simulink model "Cb_Integral_Control_Observer"  (R2025b)
settings: Solver=ode15s  StartTime=0.0  StopTime=2  RelTol=1e-9  AbsTol=1e-8
undefined symbols (not defined in the file): A11, A12, A21, A22, Bd1, Bd2, Bu1, Bu2, CA_re, CAin_re, CB_re, KH1, KH2, KH3, KH4, Ki1, Ki2, Kin1, Kin2, Kin3, Kin4, L, QH_re, Qin_V_re, T_re, Tc_re, Tin_re
settings Model: Creator=Lenovo  LastModifiedBy=Lenovo

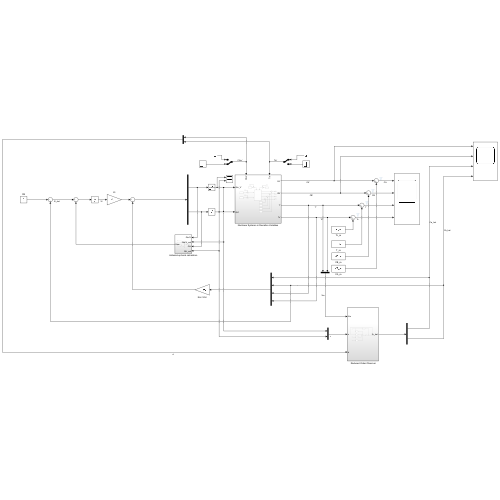
[thumbnail: Simulink's stored preview of the top-level diagram]
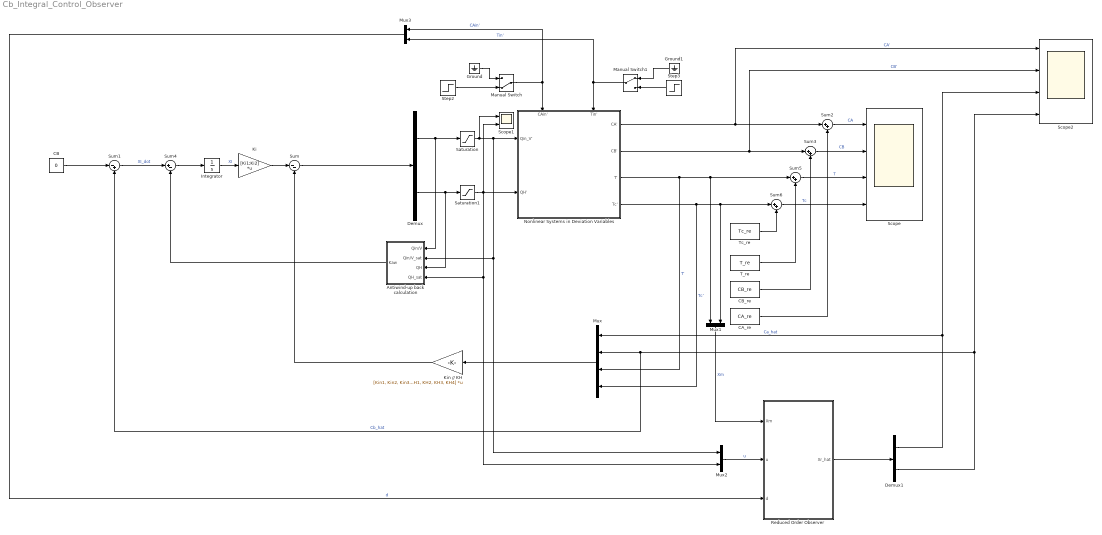
== system Cb_Integral_Control_Observer ==
  " Reduced Order Observer" : Subsystem
  Antiwind-up back calculation : Subsystem
  CA_re : Constant  Value=CA_re
  CB : Constant  Value=0
  CB_re : Constant  Value=CB_re
  Demux : Demux  Outputs=2
  Demux1 : Demux  Outputs=2
  Ground : Ground
  Ground1 : Ground
  Integrator : Integrator
  Ki : Gain  Gain=[Ki1;Ki2]  Multiplication=Matrix(K*u)
  Kin // KH : Gain  Gain=[Kin1, Kin2, Kin3, Kin4;KH1, KH2, KH3, KH4]  Multiplication=Matrix(K*u)
  Manual Switch : ManualSwitch  CurrentSetting=0
  Manual Switch1 : ManualSwitch
  Mux : Mux
  Mux1 : Mux  Inputs=2
  Mux2 : Mux  Inputs=2
  Mux3 : Mux  Inputs=2
  Nonlinear Systems in Deviation Variables : Subsystem
      settings: PortSchema="{\"entries\":[{\"content\":{\"sides\":[{\"content\":{\"connectorIds\":[\"In1\",\"In2\"]},\"type\":\"ConnectorPlacement.EquallySpacedRectSide\",\"uuid\":\"3cae5363-54ae-4836-a9af-709fc6d72947\"},{\"content\":{\"connectorIds\":[\"Out1\",\"Out2\",\"Out3\",\"Out4\"],\"side\":\"RIGHT\"},\"type\":\"ConnectorPlacement.EquallySpacedRectSide\",\"uuid\":\"ac34fbf0-7c91-43b5-9805-8d79849dc8bb\"},{\"content\":{\"connectorIds\":[\"In3\",\"In4\"],\"side\":\"TOP\"},\"type\":\"ConnectorPlacement.EquallySpacedRectSide\",\"uuid\":\"0c613297-952e-4fe2-85b3-8b705fa3960d\"}]},\"type\":\"ConnectorPlacement.EquallySpacedConnector\",\"uuid\":\"6a9d9fd9-ed65-4660-8ac2-43953dadb3cb\"}],\"packageUris\":[\"http://schema.mathworks.com/mf0/Connector/R2020b\"],\"version\":\"1.0\"}"
  Saturation : Saturate  UpperLimit=35-Qin_V_re  LowerLimit=5-Qin_V_re
  Saturation1 : Saturate  UpperLimit=0-QH_re  LowerLimit=-8500-QH_re
  Scope : Scope  NumInputPorts=4
      settings: ActiveDisplayYMinimum=-3.0170171281721987  ActiveDisplayYMaximum=25.100193696741542
  Scope1 : Scope  NumInputPorts=2
      settings: ActiveDisplayYMinimum=-4976.15012421072  ActiveDisplayYMaximum=6562.7012167590256
  Scope2 : Scope  NumInputPorts=4
      settings: ActiveDisplayYMinimum=-149.80536396754488  ActiveDisplayYMaximum=256.89603505828842  DataLoggingVariableName=ScopeData2
  Step2 : Step  Time=2  After=100  SampleTime=0
  Step3 : Step  Time=4  After=10  SampleTime=0
  Sum : Sum  Inputs=|--
  Sum1 : Sum  Inputs=|-+
  Sum{2..3,5..6} (4 alike) : Sum  Inputs=|++
  Sum4 : Sum  Inputs=|+-
  T_re : Constant  Value=T_re
  Tc_re : Constant  Value=Tc_re
  wires:
  Manual Switch1/1 -> Mux3/2, Nonlinear Systems in Deviation Variables/4(Tin')  "Tin'"
  Manual Switch/1 -> Nonlinear Systems in Deviation Variables/3(CAin'), Mux3/1  "CAin'"
  Sum/1 -> Demux/1
  Integrator/1 -> Ki/1  "XI"
  Ground/1 -> Manual Switch/1
  CB/1 -> Sum1/1
  Sum4/1 -> Integrator/1
  Demux/2 -> Antiwind-up back calculation/3(QH), Saturation1/1
  Nonlinear Systems in Deviation Variables/3(T') -> Mux/3, Sum5/1, Mux1/1  "T'"
  Nonlinear Systems in Deviation Variables/2(CB') -> Sum3/1, Scope2/2  "CB'"
  Ground1/1 -> Manual Switch1/1
  Kin // KH/1 -> Sum/2
  Mux/1 -> Kin // KH/1
  Antiwind-up back calculation/1(Kaw) -> Sum4/2
  Nonlinear Systems in Deviation Variables/4(Tc') -> Sum6/1, Mux1/2, Mux/4  "Tc'"
  Saturation1/1 -> Nonlinear Systems in Deviation Variables/2(QH'), Scope1/2, Mux2/2, Antiwind-up back calculation/4(QH_sat)
  Nonlinear Systems in Deviation Variables/1(CA') -> Scope2/1, Sum2/1  "CA'"
  Saturation/1 -> Nonlinear Systems in Deviation Variables/1(Qin_V'), Mux2/1, Antiwind-up back calculation/2(Qin/V_sat), Scope1/1
  Demux/1 -> Antiwind-up back calculation/1(Qin/V), Saturation/1
  Ki/1 -> Sum/1
  Sum1/1 -> Sum4/1  "XI_dot"
  Demux1/1 -> Scope2/3, Mux/1  "Ca_hat"
  Demux1/2 -> Sum1/2, Mux/2, Scope2/4  "Cb_hat"
  " Reduced Order Observer"/1(Xr_hat) -> Demux1/1
  Mux1/1 -> " Reduced Order Observer"/1(Xm)  "Xm"
  Mux2/1 -> " Reduced Order Observer"/2(u)  "u"
  Mux3/1 -> " Reduced Order Observer"/3(d)  "d"
  Step2/1 -> Manual Switch/2
  Step3/1 -> Manual Switch1/2
  Sum2/1 -> Scope/1  "CA"
  Sum3/1 -> Scope/2  "CB"
  Sum5/1 -> Scope/3  "T"
  Sum6/1 -> Scope/4  "Tc"
  Tc_re/1 -> Sum6/2
  T_re/1 -> Sum5/2
  CB_re/1 -> Sum3/2
  CA_re/1 -> Sum2/2

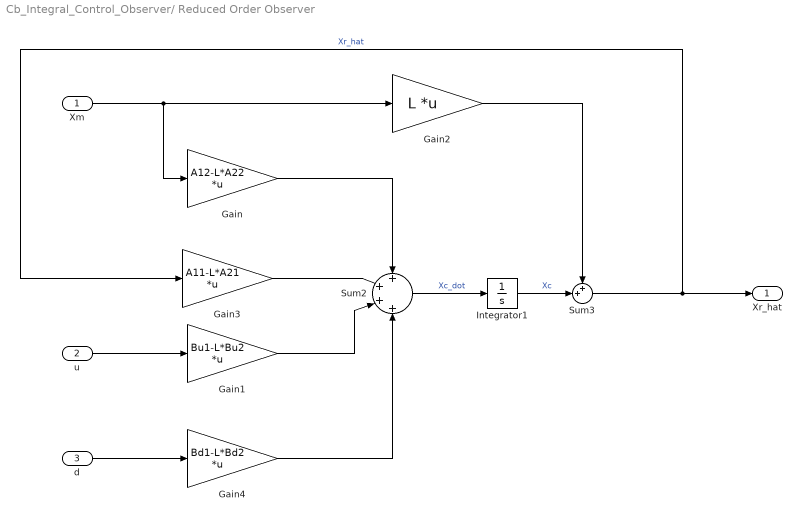
== system Cb_Integral_Control_Observer/ Reduced Order Observer ==
  Xm : Inport
  u : Inport  Port=2
  d : Inport  Port=3
  Gain : Gain  Gain=A12-L*A22  Multiplication=Matrix(K*u)
  Gain1 : Gain  Gain=Bu1-L*Bu2  Multiplication=Matrix(K*u)
  Gain2 : Gain  Gain=L  Multiplication=Matrix(K*u)
  Gain3 : Gain  Gain=A11-L*A21  Multiplication=Matrix(K*u)
  Gain4 : Gain  Gain=Bd1-L*Bd2  Multiplication=Matrix(K*u)
  Integrator1 : Integrator
  Sum2 : Sum  Inputs=+|+|+|+
  Sum3 : Sum  Inputs=++|
  Xr_hat : Outport
  wires:
  Gain1/1 -> Sum2/3
  Sum3/1 -> Gain3/1, Xr_hat/1  "Xr_hat"
  Xm/1 -> Gain/1, Gain2/1
  Integrator1/1 -> Sum3/2  "Xc"
  Gain2/1 -> Sum3/1
  Gain/1 -> Sum2/1
  Gain3/1 -> Sum2/2
  Sum2/1 -> Integrator1/1  "Xc_dot"
  u/1 -> Gain1/1
  Gain4/1 -> Sum2/4
  d/1 -> Gain4/1

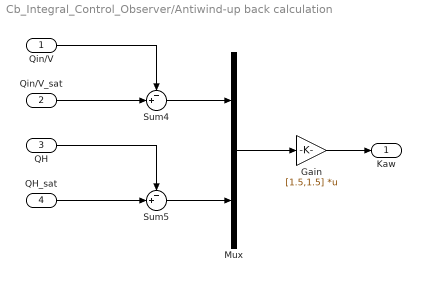
== system Cb_Integral_Control_Observer/Antiwind-up back calculation ==
  Qin/V : Inport
  Qin/V_sat : Inport  Port=2
  QH : Inport  Port=3
  QH_sat : Inport  Port=4
  Gain : Gain  Gain=[1.5,1.5]  Multiplication=Matrix(K*u)
  Mux : Mux  Inputs=2
  Sum4 : Sum  Inputs=-+|
  Sum5 : Sum  Inputs=-+|
  Kaw : Outport
  wires:
  Qin/V/1 -> Sum4/1
  Sum5/1 -> Mux/2
  Qin/V_sat/1 -> Sum4/2
  Sum4/1 -> Mux/1
  QH_sat/1 -> Sum5/2
  QH/1 -> Sum5/1
  Mux/1 -> Gain/1
  Gain/1 -> Kaw/1

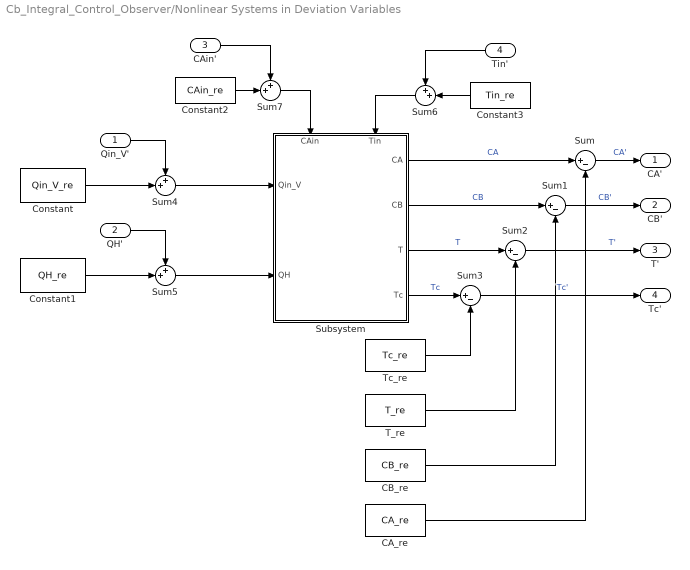
== system Cb_Integral_Control_Observer/Nonlinear Systems in Deviation Variables ==
  Qin_V' : Inport
  QH' : Inport  Port=2
  CAin' : Inport  Port=3
  Tin' : Inport  Port=4
  CA_re : Constant  Value=CA_re
  CB_re : Constant  Value=CB_re
  Constant : Constant  Value=Qin_V_re
  Constant1 : Constant  Value=QH_re
  Constant2 : Constant  Value=CAin_re
  Constant3 : Constant  Value=Tin_re
  Subsystem : Subsystem
      settings: PortSchema="{\"entries\":[{\"content\":{\"sides\":[{\"content\":{\"connectorIds\":[\"In1\",\"In2\"]},\"type\":\"ConnectorPlacement.EquallySpacedRectSide\",\"uuid\":\"3cae5363-54ae-4836-a9af-709fc6d72947\"},{\"content\":{\"connectorIds\":[\"Out1\",\"Out2\",\"Out3\",\"Out4\"],\"side\":\"RIGHT\"},\"type\":\"ConnectorPlacement.EquallySpacedRectSide\",\"uuid\":\"ac34fbf0-7c91-43b5-9805-8d79849dc8bb\"},{\"content\":{\"connectorIds\":[\"In3\",\"In4\"],\"side\":\"TOP\"},\"type\":\"ConnectorPlacement.EquallySpacedRectSide\",\"uuid\":\"0c613297-952e-4fe2-85b3-8b705fa3960d\"}]},\"type\":\"ConnectorPlacement.EquallySpacedConnector\",\"uuid\":\"6a9d9fd9-ed65-4660-8ac2-43953dadb3cb\"}],\"packageUris\":[\"http://schema.mathworks.com/mf0/Connector/R2020b\"],\"version\":\"1.0\"}"
  Sum{,1..3} (4 alike) : Sum  Inputs=|+-
  Sum{4..7} (4 alike) : Sum  Inputs=++|
  T_re : Constant  Value=T_re
  Tc_re : Constant  Value=Tc_re
  CA' : Outport
  CB' : Outport  Port=2
  T' : Outport  Port=3
  Tc' : Outport  Port=4
  wires:
  Tc_re/1 -> Sum3/2
  Subsystem/4(Tc) -> Sum3/1  "Tc"
  Subsystem/3(T) -> Sum2/1  "T"
  Sum1/1 -> CB'/1  "CB'"
  CB_re/1 -> Sum1/2
  Sum2/1 -> T'/1  "T'"
  Subsystem/1(CA) -> Sum/1  "CA"
  Sum/1 -> CA'/1  "CA'"
  Constant/1 -> Sum4/2
  T_re/1 -> Sum2/2
  Constant1/1 -> Sum5/2
  CA_re/1 -> Sum/2
  Subsystem/2(CB) -> Sum1/1  "CB"
  QH'/1 -> Sum5/1
  Sum3/1 -> Tc'/1  "Tc'"
  Qin_V'/1 -> Sum4/1
  Sum4/1 -> Subsystem/1(Qin_V)
  Sum5/1 -> Subsystem/2(QH)
  Constant3/1 -> Sum6/2
  Sum6/1 -> Subsystem/4(Tin)
  Tin'/1 -> Sum6/1
  Constant2/1 -> Sum7/2
  Sum7/1 -> Subsystem/3(CAin)
  CAin'/1 -> Sum7/1

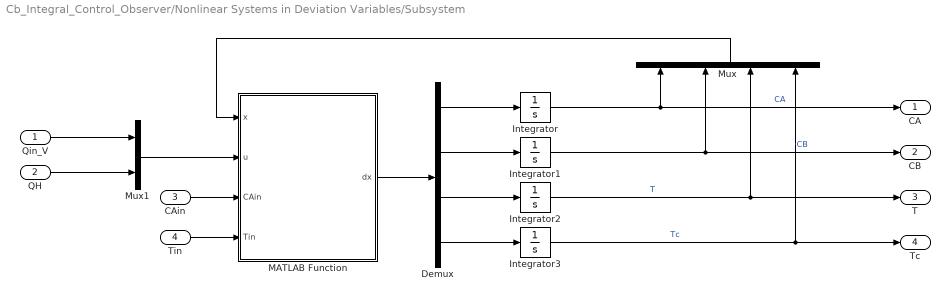
== system Cb_Integral_Control_Observer/Nonlinear Systems in Deviation Variables/Subsystem ==
  Qin_V : Inport
  QH : Inport  Port=2
  CAin : Inport  Port=3
  Tin : Inport  Port=4
  Demux : Demux
  Integrator : Integrator  InitialCondition=CA_re
  Integrator1 : Integrator  InitialCondition=CB_re
  Integrator2 : Integrator  InitialCondition=T_re
  Integrator3 : Integrator  InitialCondition=Tc_re
  MATLAB Function : MATLAB Function  TreatAsAtomicUnit=on
  Mux : Mux
  Mux1 : Mux  Inputs=2
  CA : Outport
  CB : Outport  Port=2
  T : Outport  Port=3
  Tc : Outport  Port=4
  wires:
  Demux/3 -> Integrator2/1
  Integrator1/1 -> CB/1, Mux/2  "CB"
  Integrator/1 -> CA/1, Mux/1  "CA"
  Mux/1 -> MATLAB Function/1(x)
  Integrator2/1 -> T/1, Mux/3  "T"
  Integrator3/1 -> Tc/1, Mux/4  "Tc"
  MATLAB Function/1(dx) -> Demux/1
  Demux/2 -> Integrator1/1
  Demux/4 -> Integrator3/1
  Demux/1 -> Integrator/1
  Mux1/1 -> MATLAB Function/2(u)
  Tin/1 -> MATLAB Function/4(Tin)
  QH/1 -> Mux1/2
  CAin/1 -> MATLAB Function/3(CAin)
  Qin_V/1 -> Mux1/1

== matlab function Cb_Integral_Control_Observer/Nonlinear Systems in Deviation Variables/Subsystem/MATLAB Function ==
  data: x input; u input; dx output; CAin input; Tin input
function dx = cstr_model(x, u, CAin, Tin)
dx = [0; 0; 0; 0]; 

% State variables

CA = x(1);
CB = x(2);
T  = x(3);
Tc = x(4);

% Manipulated variables
Qin_V = u(1);
QH    = u(2);

% Constants

V = 0.01;
Cp = 3.01;
den = 934.2; 
entAB = 4.2;
entBC = -11.0;
entAD = -41.85;
Ar = 0.215;
Kw = 4032;
mK = 5.0;
CpJ = 2.0;
k1_0 = 1.287e12;
k2_0 = 9.043e6;
E1 = -9758.3;
E2 = -8560.0;

% Arrhenius equations 

k1 = k1_0 * exp(E1 / (T + 273.15));
k2 = k2_0 * exp(E2 / (T + 273.15));

% Mass and energy balances

dx(1) = (Qin_V)*(CAin - CA) - k1*CA - k2*CA^2; % dCA/dt

dx(2) = -(Qin_V)*CB + k1*(CA - CB); %dCB/dt

dx(3) = (Qin_V)*(Tin - T) - (1/(den*Cp))*(k1*CA*entAB + k1*CB*entBC + k2*CA^2*entAD) + (Tc - T)*((Ar*Kw)/(den*Cp*V)); %dT/dt

dx(4) = (QH/(mK*CpJ)) + ((Ar*Kw)/(mK*CpJ))*(T - Tc); %dTc/dt

end
